simulink model "ai700_w04"  (R2024b)
settings: Solver=VariableStepAuto  StartTime=0.0  StopTime=.14  MaxStep=1e-6  RelTol=1e-3
model workspace (MAT data in the model file):
  dataset_current_command = timeseries
  dataset_current_command.Name = 'unnamed'
  dataset_current_command.DataInfo = tsdata.datametadata
  dataset_current_command.DataInfo.Interpolation = tsdata.interpolation
  dataset_current_command.DataInfo.Interpolation.Fhandle : function handle (value not decoded)
  dataset_current_command.DataInfo.Interpolation.Name = 'linear'
  dataset_current_command.TimeInfo = tsdata.timemetadata
  dataset_current_command.TimeInfo.Length = 44
  dataset_current_command.TimeInfo.DuplicateTimes = 0
  dataset_current_command.TimeInfo.Time_ = [0; 0.01; 0.039; 0.04; 0.0401666666667; 0.045; 0.0451666666667; 0.05; 0.0501666666667; 0.055; 0.0551666666667; 0.06; 0.0601666666667; 0.065; 0.0651666666667; 0.07; 0.0701666666667; 0.075; 0.0751666666667; 0.08; 0.0801666666667; 0.085; 0.0851666666667; 0.09; 0.0901666666667; 0.095; 0.0951666666667; 0.1; 0.100166666667; 0.105; 0.105166666667; 0.11; 0.110166666667; 0.115; 0.115166666667; 0.12; 0.120166666667; 0.125; 0.125166666667; 0.13; 0.130166666667; 0.135; 0.135166666667; 0.14]
  dataset_current_command.TimeInfo.Initialized = 1
  dataset_current_command.QualityInfo = tsdata.qualmetadata
  dataset_current_command.Data_ = [0; 33.3333333333; 33.3333333333; 33.3333333333; 16.6666666667; 16.6666666667; 33.3333333333; 33.3333333333; 16.6666666667; 16.6666666667; 33.3333333333; 33.3333333333; 16.6666666667; 16.6666666667; 33.3333333333; 33.3333333333; 16.6666666667; 16.6666666667; 33.3333333333; 33.3333333333; 16.6666666667; 16.6666666667; 33.3333333333; 33.3333333333; 16.6666666667; 16.6666666667; 33.3333333333; 33.3333333333; 16.6666666667; 16.6666666667; 33.3333333333; 33.3333333333; 16.6666666667; 16.6666666667; 33.3333333333; 33.3333333333; 16.6666666667; 16.6666666667; 33.3333333333; 33.3333333333; 16.6666666667; 16.6666666667; 33.3333333333; 33.3333333333]
libraries: nesl_utility x15, ee_lib x12, fl_lib x11, slpidlib x4, simulink x1
settings Model: Creator=34109  LastModifiedBy=高天宇
settings SolverCC: ZeroCrossAlgorithm=Adaptive
settings DataIOCC: SaveOutput=off  SaveTime=off
settings DebuggingCC: SignalInfNanChecking=error  IgnoredZcDiagnostic=none

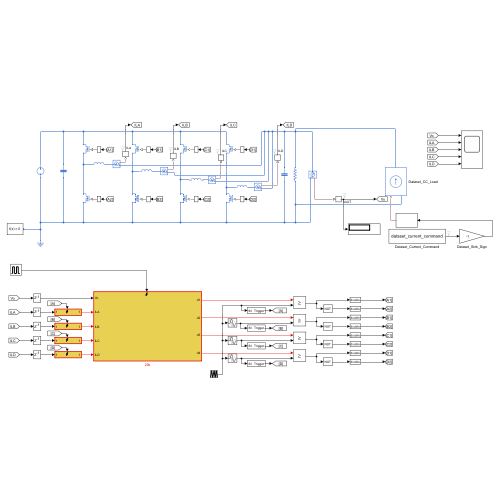
[thumbnail: Simulink's stored preview of the top-level diagram]
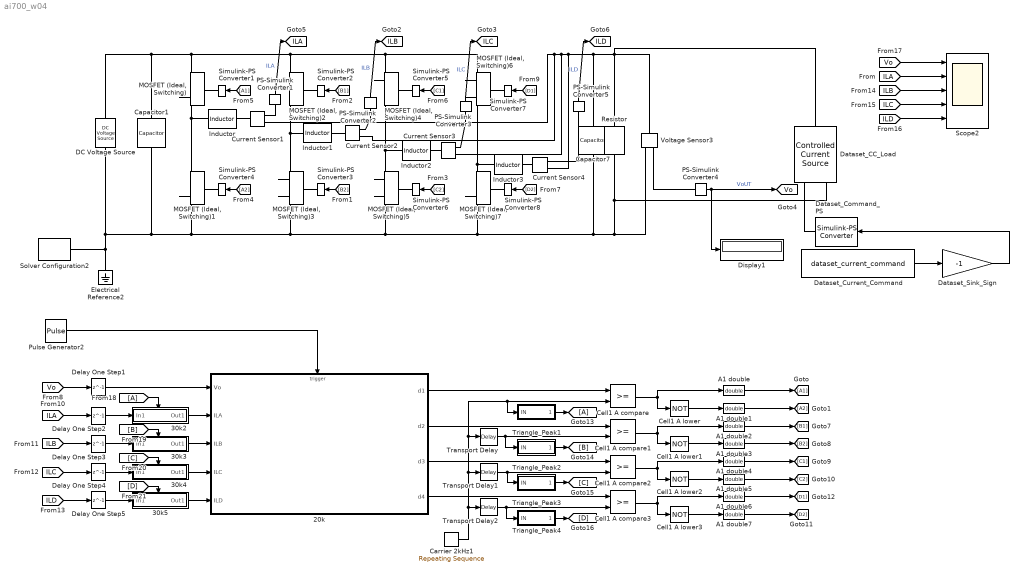
== system ai700_w04 ==
  20k : Subsystem  TreatAsAtomicUnit=on
  30k2 : Subsystem  TreatAsAtomicUnit=on
  30k3 : Subsystem  TreatAsAtomicUnit=on
  30k4 : Subsystem  TreatAsAtomicUnit=on
  30k5 : Subsystem  TreatAsAtomicUnit=on
  A1 double{,1..7} (8 alike) : DataTypeConversion  OutDataTypeStr=double  SaturateOnIntegerOverflow=off  RndMeth=Floor
  Capacitor1 : fl_lib/Electrical/Electrical Elements/Capacitor  c=180 uF  r=0.01 Ohm  g=0 1/Ohm  i_specify=off  i_priority=None  i=0 A  i_nominal_specify=off  i_nominal_value=1  i_nominal_unit=A  v_specify=off  v_priority=None  v=800 V  v_nominal_specify=off  v_nominal_value=1  v_nominal_unit=V  vc_specify=on  vc_priority=High  vc=0 V  vc_nominal_specify=off  vc_nominal_value=1  vc_nominal_unit=V
  Capacitor7 : fl_lib/Electrical/Electrical Elements/Capacitor  c=2640 uF  r=0.01 Ohm  g=0 1/Ohm  i_specify=off  i_priority=None  i=0 A  i_nominal_specify=off  i_nominal_value=1  i_nominal_unit=A  v_specify=off  v_priority=None  v=800 V  v_nominal_specify=off  v_nominal_value=1  v_nominal_unit=V  vc_specify=on  vc_priority=High  vc=0 V  vc_nominal_specify=off  vc_nominal_value=1  vc_nominal_unit=V
  Carrier 2kHz1 : simulink/Sources/Repeating Sequence  rep_seq_t=[0 1/30e3/2 1/30e3]  rep_seq_y=[0 1 0]
  Cell1 A compare{,1..3} (4 alike) : RelationalOperator  OutDataTypeStr=boolean  RndMeth=Simplest  InputSameDT=off
  Cell1 A lower{,1..3} (4 alike) : Logic  Operator=NOT  Inputs=1  AllPortsSameDT=off  OutDataTypeStr=boolean
  Current Sensor{1..4} (4 alike) : fl_lib/Electrical/Electrical Sensors/Current Sensor
  DC Voltage Source : fl_lib/Electrical/Electrical Sources/DC Voltage Source  v0=48 V
  Dataset_CC_Load : fl_lib/Electrical/Electrical Sources/Controlled Current Source
  Dataset_Command_PS : nesl_utility/Simulink-PS Converter  PhysicalDomain=network_engine_domain  SubClassName=ps_input  LeftPortType=input  RightPortType=output  PseudoPeriodic=off  Frequencies=[]  NoiseDistribution=none  NoiseParameters=[]  Unit=A  AffineConversion=off  FilteringAndDerivatives=provide  SimscapeFilterOrder=1  InputFilterTimeConstant=0.001  UdotUserProvided=0
  Dataset_Current_Command : FromWorkspace  VariableName=dataset_current_command  OutputAfterFinalValue=Holding final value
  Dataset_Sink_Sign : Gain  Gain=-1
  Delay One Step{1..5} (5 alike) : Delay  DelayLength=1
  Display1 : Display
  Electrical Reference2 : fl_lib/Electrical/Electrical Elements/Electrical Reference
  From18 : From
  Goto13 : Goto
  Inductor{,1..3} (4 alike) : ee_lib/Passive/Inductor  l=290 uH  enable_L_tol=0  L_tol=20  tol_distribution=1  nSigma=4  r=0.015 Ohm  g=1e-9 1/Ohm  enable_operating_limits=0  operating_limit_action=2  max_working_current=1 A  power_rating=1 W  fault_action=simscape.enum.assert.action.none  t_fault=1 s  i_L_specify=off  i_L_priority=High  i_L=0 A  i_L_nominal_specify=off  i_L_nominal_value=1  i_L_nominal_unit=A
  MOSFET (Ideal, Switching){,1..7} (8 alike) : ee_lib/Semiconductors & Converters/MOSFET (Ideal, Switching)  port_option=ee.enum.controlport.ps  Rds=0.01 Ohm  Goff=1e-6 1/Ohm  Vth=0.5 V  diode_param=ee.enum.converters.protectiondiode.nodynamics  diode_Vf=0.8 V  diode_Ron=0.001 Ohm  diode_Goff=1e-5 1/Ohm  diode_C=50e-9 F  diode_iRM=-235 A  diode_iF=300 A  diode_idot=-50 A/us  diode_trr_param=ee.enum.converters.diodeReverseParam.trr_factor  diode_trr_factor=3  diode_trr=15 us  diode_Qrr=1500 s*uA  ids_specify=off  ids_priority=None  ids=0 A  ids_nominal_specify=off  ids_nominal_value=1  ids_nominal_unit=A  vds_specify=off  vds_priority=None  vds=0 V  vds_nominal_specify=off  vds_nominal_value=1  vds_nominal_unit=V  vgs_specify=off  vgs_priority=None  vgs=0 V  vgs_nominal_specify=off  vgs_nominal_value=1  vgs_nominal_unit=V  thermal_loss_option=ee.enum.converters.thermalLossOption.constantvalues  Von_data=[0, 1.8, 3.2, 6, 10, 16; 0, 2, 5.5, 9.5, 15, 25] V  Tj=[298.15, 448.15] K  Iout_data=[0, 20, 40, 60, 80, 100] A  Eon_data=[0, 55.04, 124.57, 235.53, 362.12; 0, 71.25, 161.25, 304.88, 468.75] * 1e-6 J  Eoff_data=[0, 18, 30, 56.1, 76.5; 0, 22.5, 37.5, 70.13, 95.63] * 1e-6 J  Eon_data_3D=[zeros(2, 5, 3)] J  Eoff_data_3D=[zeros(2, 5, 3)] J  Tj_loss=[298.15, 448.15] K  Iout_data_loss=[0, 10, 20, 30, 40] A  tabulateWithVds=false  Vds_loss=[0, 150, 300] V  Eon_scalar=22.86e-3 J  Eoff_scalar=17.14e-3 J  Voff=300 V  Iout_scalar=600 A  useCurrentFromPreviousCycle=false  useVoltageFromPreviousCycle=false  diodeModelType=ee.enum.converters.diodeModelType.pwl  diodeTableType=ee.enum.diode.tableType.IfMat  diode_ReverseIVType=ee.enum.diode.diodeReverseIV.constant  diode_IfMat=[.07, .12, .19, 1.75, 4.24, 7.32, 11.2; .16, .3, .72, 2.14, 4.02, 6.35, 9.12] A  diode_VfMat=[.9, 1.15, 1.25, 1.5, 1.75, 2.17, 2.6, 2.85; .58, .68, .75, 1.1, 1.38, 1.77, 2.27, 2.7] V  diode_TjVec=[25, 125] degC  diode_VfVec=[.5, .7, .9, 1.3, 1.7, 2.1, 2.5] V  diode_IfVec=[.1, .2, .5, 1, 2, 4, 7, 10] A  diode_IrMat=[1e-06, 2e-06, 5e-06, 1e-05, 2.5e-05, 5e-05, .0001; 2e-06, 5e-06, 1e-05, 4e-05, 8e-05, .0002, .0005] A  diode_VrMat=[10, 100, 200, 250, 300, 325, 350; 10, 70, 160, 220, 270, 300, 320] V  diode_VrVec=[10, 20, 40, 50, 70, 80, 100] V  diode_IrVec=[1e-06, 2e-06, 5e-06, 1e-05, 2e-05, 5e-05, .0001] A  diode_Vr=-600 V  diode_Ls=150 nH  diode_Erec=0.03 J  diode_rec_loss_model=ee.enum.diode.reverseRecoveryModel.fixed  diode_ErecVal=0 J  diode_scaleWithIandV=true  diode_ErecMat=zeros(2, 3) J  diode_TjrecVec=[298.15, 398.15] K  diode_IfrecVec=[.1, 1, 10] A  diode_IrecVal=10 A  diode_VrecVal=10 V  diode_tFilter=1 / 1000 / 100 s  separateThermalPortForDiode=false  thermal_network_parameterization=ee.enum.thermalNetworkTopology.external  Rth=[.03, .2] K/W  Rth_Cauer=[.03, .1, .2] K/W  Rth_Foster=[.03, .2] K/W  thermal_mass_parameterization=ee.enum.thermalNetwork.timeconstant  thermal_mass=[3, 25] J/K  thermal_mass_Cauer=[3, 10, 25] J/K  thermal_mass_Foster=[33, 50] J/K  thermal_time_constant=[.1, 5] s  thermal_time_constant_Cauer=[.1, 1, 5] s  thermal_time_constant_Foster=[1, 10] s  thermal_mass_initial_temperatures=[25, 25] degC  thermal_mass_initial_temperatures_Cauer=[25, 25, 25] degC  junction_thermal_mass=0.1 J/K  Tvec_initial_Foster=[25, 25, 25, 25] degC  RthDiode=[.03, .2] K/W  RthCauerDiode=[.03, .1, .2] K/W  RthFosterDiode=[.03, .2] K/W  thermalMassDiode=[3, 25] J/K  thermalMassCauerDiode=[3, 10, 25] J/K  thermalMassFosterDiode=[33, 50] J/K  thermalTauDiode=[.1, 5] s  thermalTauCauerDiode=[.1, 1, 5] s  thermalTauFosterDiode=[1, 10] s  thermalMassInitTempDiode=[25, 25] degC  thermalMassInitTempCauerDiode=[25, 25, 25] degC  junctionthermalMassDiode=0.1 J/K  TVecInitialFosterDiode=[25, 25, 25, 25] degC  no_thermal_network=0  mosfet_junction_temperature_specify=off  mosfet_junction_temperature_priority=None  mosfet_junction_temperature=25 degC  mosfet_junction_temperature_nominal_specify=off  mosfet_junction_temperature_nominal_value=1  mosfet_junction_temperature_nominal_unit=degC  diode_junction_temperature_specify=off  diode_junction_temperature_priority=None  diode_junction_temperature=25 degC  diode_junction_temperature_nominal_specify=off  diode_junction_temperature_nominal_value=1  diode_junction_temperature_nominal_unit=degC  Qj_specify=off  Qj_priority=None  Qj=0 W  Qj_nominal_specify=off  Qj_nominal_value=1  Qj_nominal_unit=W  accumulatedSwitchingLosses_specify=off  accumulatedSwitchingLosses_priority=None  accumulatedSwitchingLosses=0 J
  PS-Simulink Converter{1..5} (5 alike) : nesl_utility/PS-Simulink Converter  PhysicalDomain=network_engine_domain  SubClassName=ps_output  LeftPortType=input  RightPortType=output  PseudoPeriodic=off  Frequencies=[]  VectorFormat=inherit  Unit=inherit  AffineConversion=off
  Pulse Generator2 : DiscretePulseGenerator  PulseType=Time based  Period=1/30000  PulseWidth=5
  Resistor : fl_lib/Electrical/Electrical Elements/Resistor  R=1e9 Ohm  i_specify=off  i_priority=None  i=0 A  i_nominal_specify=off  i_nominal_value=1  i_nominal_unit=A  v_specify=off  v_priority=None  v=0 V  v_nominal_specify=off  v_nominal_value=1  v_nominal_unit=V
  Scope2 : Scope  NumInputPorts=5
  Simulink-PS Converter{1..8} (8 alike) : nesl_utility/Simulink-PS Converter  PhysicalDomain=network_engine_domain  SubClassName=ps_input  LeftPortType=input  RightPortType=output  PseudoPeriodic=off  Frequencies=[]  NoiseDistribution=none  NoiseParameters=[]  Unit=1  AffineConversion=off  FilteringAndDerivatives=provide  SimscapeFilterOrder=1  InputFilterTimeConstant=0.001  UdotUserProvided=0
  Solver Configuration2 : nesl_utility/Solver Configuration  PhysicalDomain=network_engine_domain  SubClassName=solver  LeftPortType=input  RightPortType=generic  Tones=[]  Harmonics=[]  SimulateNoise=off  Profile=off  UseLocalSampling=off  EnableSwitchedLinearOptims=on  FrequencyDomain=off  UseCCode=off  RelTol=0.001  AbsTol=1e-06  MinStep=1e-09  ToWorkspace=off  RevertToSquareIcSolve=off  NumHomotopyIterations=100  PhasorMode=off  PhasorModeNumHarmonics=1  ConsistencySolver=NEWTON_XTOL_AFTER_FTOL  IndexReductionMethod=DerivativeReplacement  DoDC=off  ResidualTolerance=1e-09  ConsistencyTolSource=GLOBAL  ConsistencyAbsTol=0.001  ConsistencyRelTol=0.001  ConsistencyTolFactor=0.001  UseLocalSolver=on  LocalSolverChoice=NE_BACKWARD_EULER_ADVANCER  ResolveIndetEquations=on  FunctionEvalNumThread=1  LocalSolverSampleTime=1e-7  DoFixedCost=off  MaxNonlinIter=3  MaxModeIter=2  ComputeImpulses=off  ImpulseIterations=2  LinearAlgebra=auto  LinearAlgebraNumThread=0  EquationFormulation=NE_TIME_EF  DelaysMemoryBudget=1024  AutomaticFiltering=on  FilteringTimeConstant=0.001  PartitionStorageMethod=AS_NEEDED  PartitionMemoryBudget=1024  PartitionMethod=ROBUST  MultibodyUseLocalSolver=off  MultibodyLocalSolverChoice=ODE1  MultibodyLocalSolverSampleTime=0.001
  Transport Delay : TransportDelay  DelayTime=1/30e3/4
  Transport Delay1 : TransportDelay  DelayTime=1/30e3/4*2
  Transport Delay2 : TransportDelay  DelayTime=1/30e3/4*3
  Triangle_Peak1 : Subsystem
  Triangle_Peak2 : Subsystem
  Triangle_Peak3 : Subsystem
  Triangle_Peak4 : Subsystem
  Voltage Sensor3 : fl_lib/Electrical/Electrical Sensors/Voltage Sensor
  tag scope: ILA=global, ILB=global, ILC=global, ILD=global, Vo=global
  wires:
  PS-Simulink Converter1/1 -> [ILA]  "ILA"
  Pulse Generator2/1 -> 20k/Trigger
  [A2] -> Simulink-PS Converter4/1
  [A1] -> Simulink-PS Converter1/1
  PS-Simulink Converter4/1 -> [Vo], Display1/1  "VoUT"
  [B1] -> Simulink-PS Converter2/1
  [B2] -> Simulink-PS Converter3/1
  [C2] -> Simulink-PS Converter6/1
  [C1] -> Simulink-PS Converter5/1
  [D1] -> Simulink-PS Converter7/1
  [D2] -> Simulink-PS Converter8/1
  PS-Simulink Converter2/1 -> [ILB]  "ILB"
  PS-Simulink Converter3/1 -> [ILC]  "ILC"
  PS-Simulink Converter5/1 -> [ILD]  "ILD"
  [Vo] -> Scope2/1
  [ILA] -> Scope2/2
  [ILB] -> Scope2/3
  [ILC] -> Scope2/4
  [ILD] -> Scope2/5
  Dataset_Current_Command/1 -> Dataset_Sink_Sign/1
  Dataset_Sink_Sign/1 -> Dataset_Command_PS/1
  Delay One Step5/1 -> 30k5/1(In1)
  Delay One Step3/1 -> 30k3/1(In1)
  30k5/1(Out1) -> 20k/5(ILD)
  30k4/1(Out1) -> 20k/4(ILC)
  [D] -> 30k5/Trigger
  Delay One Step2/1 -> 30k2/1(In1)
  From18/1 -> 30k2/Trigger
  [ILA] -> Delay One Step2/1
  [C] -> 30k4/Trigger
  30k2/1(Out1) -> 20k/2(ILA)
  Delay One Step4/1 -> 30k4/1(In1)
  [B] -> 30k3/Trigger
  [ILD] -> Delay One Step5/1
  [ILC] -> Delay One Step4/1
  30k3/1(Out1) -> 20k/3(ILB)
  [Vo] -> Delay One Step1/1
  [ILB] -> Delay One Step3/1
  Delay One Step1/1 -> 20k/1(Vo)
  Transport Delay2/1 -> Triangle_Peak4/1(IN), Cell1 A compare3/2
  Transport Delay1/1 -> Triangle_Peak3/1(IN), Cell1 A compare2/2
  Triangle_Peak3/1(Trigger) -> [C]
  Cell1 A lower/1 -> A1 double1/1
  Cell1 A lower3/1 -> A1 double7/1
  Triangle_Peak2/1(Trigger) -> [B]
  20k/3(d3) -> Cell1 A compare2/1
  A1 double7/1 -> [D2]
  A1 double5/1 -> [C2]
  Cell1 A compare2/1 -> A1 double4/1, Cell1 A lower2/1
  Carrier 2kHz1/1 -> Triangle_Peak1/1(IN), Cell1 A compare/2, Transport Delay/1, Transport Delay1/1, Transport Delay2/1
  20k/2(d2) -> Cell1 A compare1/1
  Cell1 A compare3/1 -> Cell1 A lower3/1, A1 double6/1
  A1 double/1 -> [A1]
  A1 double6/1 -> [D1]
  Triangle_Peak4/1(Trigger) -> [D]
  A1 double3/1 -> [B2]
  Cell1 A compare1/1 -> Cell1 A lower1/1, A1 double2/1
  A1 double4/1 -> [C1]
  Cell1 A lower1/1 -> A1 double3/1
  20k/4(d4) -> Cell1 A compare3/1
  Cell1 A compare/1 -> A1 double/1, Cell1 A lower/1
  Triangle_Peak1/1(Trigger) -> Goto13/1
  A1 double2/1 -> [B1]
  Transport Delay/1 -> Triangle_Peak2/1(IN), Cell1 A compare1/2
  Cell1 A lower2/1 -> A1 double5/1
  20k/1(d1) -> Cell1 A compare/1
  A1 double1/1 -> [A2]
  connections:
  Voltage Sensor3/RConn2 -- "MOSFET (Ideal, Switching)3"/RConn2 -- Electrical Reference2/LConn1 -- Solver Configuration2/RConn1 -- DC Voltage Source/RConn1 -- Capacitor1/RConn1 -- "MOSFET (Ideal, Switching)1"/RConn2 -- "MOSFET (Ideal, Switching)5"/RConn2 -- "MOSFET (Ideal, Switching)7"/RConn2 -- Capacitor7/RConn1 -- Resistor/RConn1 -- Dataset_CC_Load/RConn2
  "MOSFET (Ideal, Switching)"/LConn1 -- Simulink-PS Converter1/RConn1
  PS-Simulink Converter4/LConn1 -- Voltage Sensor3/RConn1
  "MOSFET (Ideal, Switching)1"/LConn1 -- Simulink-PS Converter4/RConn1
  Resistor/LConn1 -- Dataset_CC_Load/LConn1 -- Current Sensor4/RConn2 -- Current Sensor3/RConn2 -- Current Sensor2/RConn2 -- Current Sensor1/RConn2 -- Capacitor7/LConn1 -- Voltage Sensor3/LConn1
  PS-Simulink Converter1/LConn1 -- Current Sensor1/RConn1
  "MOSFET (Ideal, Switching)3"/LConn1 -- Simulink-PS Converter3/RConn1
  "MOSFET (Ideal, Switching)2"/LConn1 -- Simulink-PS Converter2/RConn1
  "MOSFET (Ideal, Switching)3"/RConn1 -- Inductor1/LConn1 -- "MOSFET (Ideal, Switching)2"/RConn2
  "MOSFET (Ideal, Switching)4"/LConn1 -- Simulink-PS Converter5/RConn1
  "MOSFET (Ideal, Switching)5"/LConn1 -- Simulink-PS Converter6/RConn1
  "MOSFET (Ideal, Switching)7"/LConn1 -- Simulink-PS Converter8/RConn1
  "MOSFET (Ideal, Switching)6"/LConn1 -- Simulink-PS Converter7/RConn1
  DC Voltage Source/LConn1 -- Capacitor1/LConn1 -- "MOSFET (Ideal, Switching)6"/RConn1 -- "MOSFET (Ideal, Switching)4"/RConn1 -- "MOSFET (Ideal, Switching)2"/RConn1 -- "MOSFET (Ideal, Switching)"/RConn1
  "MOSFET (Ideal, Switching)5"/RConn1 -- Inductor2/LConn1 -- "MOSFET (Ideal, Switching)4"/RConn2
  "MOSFET (Ideal, Switching)6"/RConn2 -- Inductor3/LConn1 -- "MOSFET (Ideal, Switching)7"/RConn1
  "MOSFET (Ideal, Switching)"/RConn2 -- Inductor/LConn1 -- "MOSFET (Ideal, Switching)1"/RConn1
  Inductor/RConn1 -- Current Sensor1/LConn1
  Inductor1/RConn1 -- Current Sensor2/LConn1
  PS-Simulink Converter2/LConn1 -- Current Sensor2/RConn1
  PS-Simulink Converter3/LConn1 -- Current Sensor3/RConn1
  Inductor2/RConn1 -- Current Sensor3/LConn1
  Current Sensor4/LConn1 -- Inductor3/RConn1
  PS-Simulink Converter5/LConn1 -- Current Sensor4/RConn1
  Dataset_Command_PS/RConn1 -- Dataset_CC_Load/RConn1

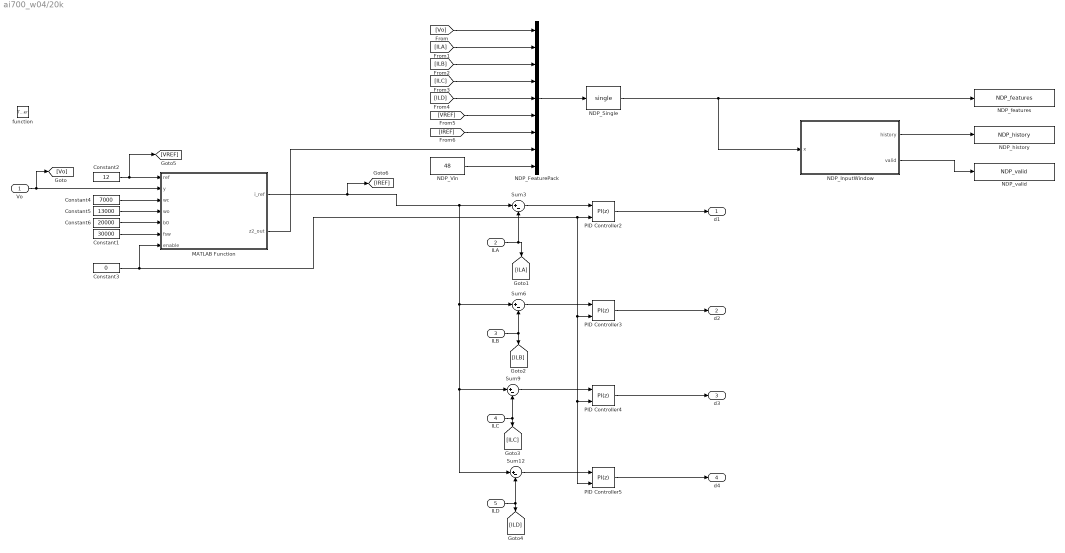
== system ai700_w04/20k ==
  Vo : Inport
  ILA : Inport  Port=2
  ILB : Inport  Port=3
  ILC : Inport  Port=4
  ILD : Inport  Port=5
  function : TriggerPort  VariantControl=(inherit)  InitialTriggerSignalState=zero
  Constant1 : Constant  Value=30000
  Constant2 : Constant  Value=12
  Constant3 : Constant  Value=0
  Constant4 : Constant  Value=7000
  Constant5 : Constant  Value=13000
  Constant6 : Constant  Value=20000
  MATLAB Function : MATLAB Function  TreatAsAtomicUnit=on
  NDP_FeaturePack : Mux  Inputs=9
  NDP_InputWindow : MATLAB Function  TreatAsAtomicUnit=on
  NDP_Single : DataTypeConversion  OutDataTypeStr=single  SaturateOnIntegerOverflow=off  RndMeth=Floor
  NDP_Vin : Constant  Value=48
  NDP_features : ToWorkspace  VariableName=NDP_features  SaveFormat=Timeseries  SampleTime=-1
  NDP_history : ToWorkspace  VariableName=NDP_history  SaveFormat=Timeseries  SampleTime=-1
  NDP_valid : ToWorkspace  VariableName=NDP_valid  SaveFormat=Timeseries  SampleTime=-1
  PID Controller{2..5} (4 alike) : slpidlib/PID Controller  Controller=PI  Form=Parallel  TimeDomain=Discrete-time  UseExternalTs=off  SampleTime=-1  IntegratorMethod=Forward Euler  FilterMethod=Forward Euler  ControllerParametersSource=internal  P=0.02  I=0.00025000000000000001  UseKiTs=on  D=0  UseExternalDerivativeSource=off  N=100  UseFilter=on  TunerSelectOption=Transfer Function Based (PID Tuner App)  InitialConditionSource=internal  InitialConditionForIntegrator=0.05  InitialConditionForFilter=0  DifferentiatorICPrevScaledInput=0  ExternalReset=either  TrackingMode=off  Kt=1  LimitOutput=on  SatLimitsSource=internal  UpperSaturationLimit=0.95  LowerSaturationLimit=0.05  LinearizeAsGain=on  AntiWindupMode=clamping  Kb=1  LimitIntegrator=off  UpperIntegratorSaturationLimit=inf  LowerIntegratorSaturationLimit=-inf  POutMin=[]  POutMax=[]  IOutMin=[]  IOutMax=[]  DOutMin=[]  DOutMax=[]  NOutMin=[]  NOutMax=[]  SumOutMin=[]  SumOutMax=[]  SaturationOutMin=[]  SaturationOutMax=[]  PParamMin=[]  PParamMax=[]  IParamMin=[]  IParamMax=[]  DParamMin=[]  DParamMax=[]  NParamMin=[]  NParamMax=[]  KbParamMin=[]  KbParamMax=[]  KtParamMin=[]  KtParamMax=[]  KbOutMin=[]  KbOutMax=[]  KtOutMin=[]  KtOutMax=[]  IntegratorOutMin=[]  IntegratorOutMax=[]  FilterOutMin=[]  FilterOutMax=[]  SumI1OutMin=[]  SumI1OutMax=[]  SumI2OutMin=[]  SumI2OutMax=[]  SumI3OutMin=[]  SumI3OutMax=[]  SumI4OutMin=[]  SumI4OutMax=[]  SumDOutMin=[]  SumDOutMax=[]  DifferentiatorOutMin=[]  DifferentiatorOutMax=[]  FilterDiffOutCoefMin=[]  FilterDiffOutCoefMax=[]  ReciprocalOutMin=[]  ReciprocalOutMax=[]  SumDenOutMin=[]  SumDenOutMax=[]  SumNumOutMin=[]  SumNumOutMax=[]  DivideOutMin=[]  DivideOutMax=[]  UdiffTsProdOutMin=[]  UdiffTsProdOutMax=[]  NTsProdOutMin=[]  NTsProdOutMax=[]  UintegralTsProdOutMin=[]  UintegralTsProdOutMax=[]  UngainTsProdOutMin=[]  UngainTsProdOutMax=[]  ClampingZeroOutDataTypeStr=Inherit: Inherit via back propagation  ClampingZeroOutMin=[]  ClampingZeroOutMax=[]  FilterDenConstantOutDataTypeStr=Inherit: Inherit via back propagation  FilterDenConstantOutMin=[]  FilterDenConstantOutMax=[]  PCopyOutDataTypeStr=Inherit: Inherit via back propagation  PCopyOutMin=[]  PCopyOutMax=[]  NCopyOutDataTypeStr=Inherit: Inherit via back propagation  NCopyOutMin=[]  NCopyOutMax=[]  IntegratorContinuousStateAttributes=''  IntegratorStateMustResolveToSignalObject=off  IntegratorRTWStateStorageClass=Auto  FilterContinuousStateAttributes=''  FilterStateMustResolveToSignalObject=off  FilterRTWStateStorageClass=Auto  ParallelPVariant=InternalParameters  IdealPVariant=Disabled  IVariant=InternalParameters  DVariant=Disabled  IntegratorVariant=Discrete  SatVariant=Enabled  AWVariant=DiscClampingParallel  PCopyVariant=Disabled  TRVariant=Disabled  FdbkBlocksVariant=Forward  IdealPFdbkVariant=Disabled  SatFdbkVariant=Disabled  DerivativeFilterVariant=Disabled  NVariant=Disabled  NCopyVariant=Disabled_SignalSpec  FilterICVariant=Disabled  IntegratorICVariant=InternalICs  ExternalResetVariant=ExternalReset  TRSumVariant=Passthrough  SumFdbkVariant=Disabled  SumVariant=Sum_PI  TsampFilterVariant=InternalTs  TsampNgainVariant=Passthrough  TsampIntegralVariant=Disabled_SignalSpec  ExternalSaturationOutDataTypeStr=Inherit: Same as second input  DerivativeSourceVariant=Disabled  PreIntVariant=InternalPreInt
  Sum{3,6,9,12} (4 alike) : Sum  Inputs=|+-
  d1 : Outport
  d2 : Outport  Port=2
  d3 : Outport  Port=3
  d4 : Outport  Port=4
  wires:
  MATLAB Function/1(i_ref) -> [IREF], Sum12/1, Sum9/1, Sum6/1, Sum3/1
  Constant1/1 -> MATLAB Function/6(fsw)
  ILB/1 -> [ILB], Sum6/2
  Constant3/1 -> MATLAB Function/7(enable), PID Controller5/2, PID Controller4/2, PID Controller3/2, PID Controller2/2
  Sum9/1 -> PID Controller4/1
  Sum12/1 -> PID Controller5/1
  PID Controller5/1 -> d4/1
  Constant2/1 -> [VREF], MATLAB Function/1(ref)
  Constant6/1 -> MATLAB Function/5(b0)
  PID Controller3/1 -> d2/1
  Vo/1 -> [Vo], MATLAB Function/2(y)
  Constant4/1 -> MATLAB Function/3(wc)
  Sum3/1 -> PID Controller2/1
  ILA/1 -> [ILA], Sum3/2
  ILC/1 -> [ILC], Sum9/2
  ILD/1 -> [ILD], Sum12/2
  PID Controller4/1 -> d3/1
  Constant5/1 -> MATLAB Function/4(wo)
  Sum6/1 -> PID Controller3/1
  PID Controller2/1 -> d1/1
  MATLAB Function/2(z2_out) -> NDP_FeaturePack/8
  NDP_Vin/1 -> NDP_FeaturePack/9
  NDP_FeaturePack/1 -> NDP_Single/1
  NDP_Single/1 -> NDP_features/1, NDP_InputWindow/1(x)
  NDP_InputWindow/1(history) -> NDP_history/1
  NDP_InputWindow/2(valid) -> NDP_valid/1
  [Vo] -> NDP_FeaturePack/1
  [ILA] -> NDP_FeaturePack/2
  [ILB] -> NDP_FeaturePack/3
  [ILC] -> NDP_FeaturePack/4
  [ILD] -> NDP_FeaturePack/5
  [VREF] -> NDP_FeaturePack/6
  [IREF] -> NDP_FeaturePack/7

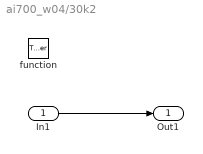
== system ai700_w04/30k2 ==
  In1 : Inport
  function : TriggerPort  VariantControl=(inherit)  InitialTriggerSignalState=zero
  Out1 : Outport
  wires:
  In1/1 -> Out1/1

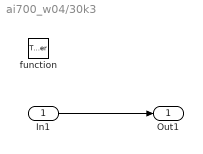
== system ai700_w04/30k3 ==
  In1 : Inport
  function : TriggerPort  VariantControl=(inherit)  InitialTriggerSignalState=zero
  Out1 : Outport
  wires:
  In1/1 -> Out1/1

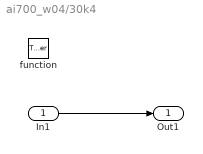
== system ai700_w04/30k4 ==
  In1 : Inport
  function : TriggerPort  VariantControl=(inherit)  InitialTriggerSignalState=zero
  Out1 : Outport
  wires:
  In1/1 -> Out1/1

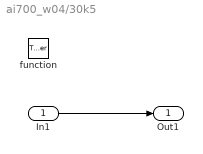
== system ai700_w04/30k5 ==
  In1 : Inport
  function : TriggerPort  VariantControl=(inherit)  InitialTriggerSignalState=zero
  Out1 : Outport
  wires:
  In1/1 -> Out1/1

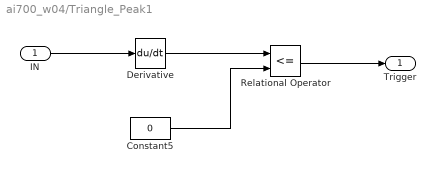
== system ai700_w04/Triangle_Peak1 ==
  IN : Inport
  Constant5 : Constant  Value=0
  Derivative : Derivative
  Relational Operator : RelationalOperator  Operator=<=  OutDataTypeStr=boolean  RndMeth=Simplest  InputSameDT=off
  Trigger : Outport
  wires:
  Relational Operator/1 -> Trigger/1
  Derivative/1 -> Relational Operator/1
  Constant5/1 -> Relational Operator/2
  IN/1 -> Derivative/1

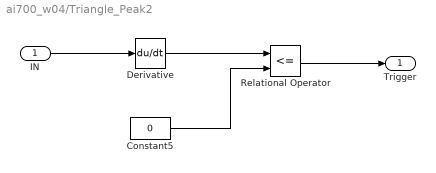
== system ai700_w04/Triangle_Peak2 ==
  IN : Inport
  Constant5 : Constant  Value=0
  Derivative : Derivative
  Relational Operator : RelationalOperator  Operator=<=  OutDataTypeStr=boolean  RndMeth=Simplest  InputSameDT=off
  Trigger : Outport
  wires:
  IN/1 -> Derivative/1
  Constant5/1 -> Relational Operator/2
  Derivative/1 -> Relational Operator/1
  Relational Operator/1 -> Trigger/1

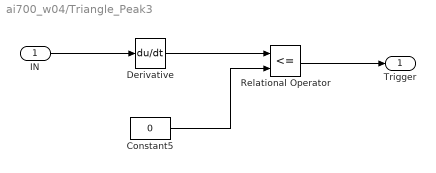
== system ai700_w04/Triangle_Peak3 ==
  IN : Inport
  Constant5 : Constant  Value=0
  Derivative : Derivative
  Relational Operator : RelationalOperator  Operator=<=  OutDataTypeStr=boolean  RndMeth=Simplest  InputSameDT=off
  Trigger : Outport
  wires:
  Relational Operator/1 -> Trigger/1
  Derivative/1 -> Relational Operator/1
  Constant5/1 -> Relational Operator/2
  IN/1 -> Derivative/1

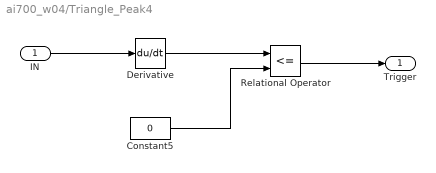
== system ai700_w04/Triangle_Peak4 ==
  IN : Inport
  Constant5 : Constant  Value=0
  Derivative : Derivative
  Relational Operator : RelationalOperator  Operator=<=  OutDataTypeStr=boolean  RndMeth=Simplest  InputSameDT=off
  Trigger : Outport
  wires:
  IN/1 -> Derivative/1
  Constant5/1 -> Relational Operator/2
  Derivative/1 -> Relational Operator/1
  Relational Operator/1 -> Trigger/1

== matlab function ai700_w04/20k/NDP_InputWindow ==
  data: x input; history output; valid output
function [history,valid] = ndp_window(x)
%#codegen
% One update per enclosing controller trigger. Oldest sample first.
persistent buf count
if isempty(buf)
    buf=zeros(9,8,'single');
    count=uint8(0);
end
buf(:,1:7)=buf(:,2:8);
buf(:,8)=x;
if count<uint8(8), count=count+uint8(1); end
history=reshape(buf,72,1);
valid=count==uint8(8);
end

== matlab function ai700_w04/20k/MATLAB Function ==
  data: ref input; i_ref output; y input; wc input; wo input; b0 input; fsw input; enable input; z2_out output
function [i_ref,z2_out] = Voltage_ADRC(ref, y, wc, wo, b0, fsw, enable)
%#codegen
% 一阶 LADRC 电压外环，输出电感电流给定 i_ref（A）。
% ref、y：目标电压和实测电压（V）。
% wc：电压环控制带宽；wo：ESO 观测器带宽（rad/s）。
% b0：电流对电压变化速度的标称作用系数。
% enable = 1：复位；enable = 0：运行。

persistent z1 z2 u_prev
% z1：输出电压估计值。
% z2：负载变化、参数误差等因素的总扰动估计值。
% u_prev：上一采样周期已限幅的电流给定。

ref_s = single(ref);
y_s   = single(y);
wc_s  = single(wc);
wo_s  = single(wo);
b0_s  = single(b0);
Ts    = single(1) / single(fsw);
Imax  = single(40);
zero  = single(0);

if isempty(z1)
    % 首次运行时，从当前实测电压开始估计。
    z1 = y_s;
    z2 = zero;
    u_prev = zero;
end

if enable == 1
    % 停机期间持续清除扰动估计，并让电压估计跟踪实测值。
    % 再次使能时，从当前电压开始控制。
    z1 = y_s;
    z2 = zero;
    u_prev = zero;
    i_ref = double(zero);
else
    % ESO：用实测电压与估计电压的差值修正状态估计。
    e = y_s - z1;
    z1_old = z1;
    z1 = z1_old + Ts*(z2 + b0_s*u_prev + single(2)*wo_s*e);
    z2 = z2 + Ts*(wo_s*wo_s*e);

    % wc*(ref-z1) 调节电压误差，减去 z2 补偿估计出的扰动。
    raw = (wc_s*(ref_s - z1) - z2) / b0_s;

    % 限制电流给定，避免外环要求超出允许范围的电流。
    cmd = min(max(raw, -Imax), Imax);

    % 保存本周期给定，供下一周期 ESO 更新使用。
    u_prev = cmd;
    i_ref = double(cmd);
end
z2_out = double(z2);
end
